simulink model "ACC_System"  (R2026b)
settings: Solver=VariableStepAuto  StopTime=30  FixedStep=0.01
settings Model: Creator=Ahmed  LastModifiedBy=Ahmed
settings RTWCC: GenCodeOnly=on  GenerateReport=on  LaunchReport=on

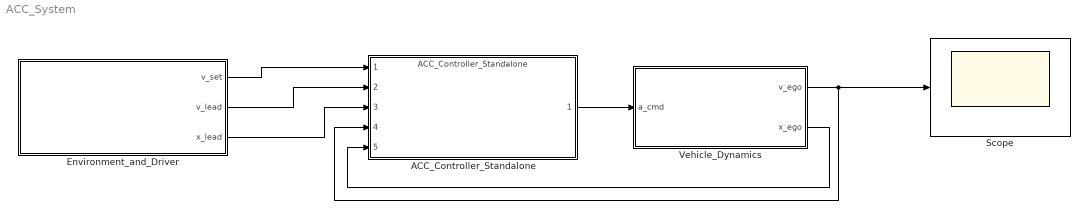
== system ACC_System ==
  ACC_Controller_Standalone : ModelReference  ModelNameDialog=ACC_Controller_Standalone.slx  SimulationMode=Normal  ModelReferenceVersion=1.2
  Environment_and_Driver : Subsystem
  Scope : Scope
      settings: ActiveDisplayYMinimum=7.8768012136808956  ActiveDisplayYMaximum=29.10878907687195
  Vehicle_Dynamics : Subsystem
  wires:
  Environment_and_Driver/2(v_lead) -> ACC_Controller_Standalone/2
  Environment_and_Driver/3(x_lead) -> ACC_Controller_Standalone/3
  ACC_Controller_Standalone/1 -> Vehicle_Dynamics/1(a_cmd)
  Vehicle_Dynamics/2(x_ego) -> ACC_Controller_Standalone/5
  Vehicle_Dynamics/1(v_ego) -> ACC_Controller_Standalone/4, Scope/1
  Environment_and_Driver/1(v_set) -> ACC_Controller_Standalone/1

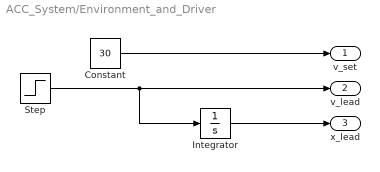
== system ACC_System/Environment_and_Driver ==
  Constant : Constant  Value=30
  Integrator : Integrator  InitialCondition=40
  Step : Step  Time=15  InitialValue=20  FinalValue=10  SampleTime=0
  v_set : Outport
  v_lead : Outport  Port=2
  x_lead : Outport  Port=3
  wires:
  Constant/1 -> v_set/1
  Step/1 -> Integrator/1, v_lead/1
  Integrator/1 -> x_lead/1

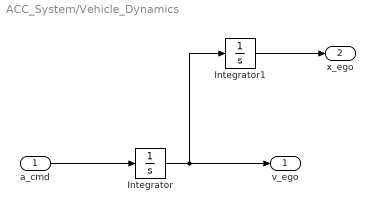
== system ACC_System/Vehicle_Dynamics ==
  a_cmd : Inport
  Integrator : Integrator  InitialCondition=10  LimitOutput=on  UpperSaturationLimit=50  LowerSaturationLimit=0
  Integrator1 : Integrator
  v_ego : Outport
  x_ego : Outport  Port=2
  wires:
  a_cmd/1 -> Integrator/1
  Integrator1/1 -> x_ego/1
  Integrator/1 -> Integrator1/1, v_ego/1
